simulink library "sm_wheel_loader_lib"  (R2025a)
settings: Solver=VariableStepAuto  StartTime=0.0  StopTime=10.0  RelTol=1e-3
undefined symbols (not defined in the file): AToTOrificeVector, BiPOrificeVector, boomHEArea, boomREArea, BToTOrificeVector, fluids, GRake, GToothL, GToothR, HMPST, HydFcnParams, logLoad, Position, PToAOrificeVector, PToBOrificeVector, RakeL, RakeR, testInput, Wheel_Loader, X, Y, Z
libraries: sm_lib x694, fl_lib x183, nesl_utility x74, SimscapeFluids_lib x62, sdl_lib x25, cvt_components_lib x25, simulink_extras x5, $bdroot x4, wheel_loader_contact_lib x4, ee_lib x2, SignalEditorBlockLib x1, batteryecm_lib x1
(part 14 of 26)

== system sm_wheel_loader_lib/Wheel Loader Vehicle/Load/Log/Bin ==
  Brick A : sm_lib/Body Elements/Brick Solid  BrickDimensions="[0.1 5.5  1]"  BrickDimensionsUnits=m  ExportEntireGeometry=on  InertiaType=CalculateFromGeometry  BasedOnType=Density  Density=1000  DensityUnits=kg/m^3  Mass=1  MassUnits=kg  CenterOfMass=[0 0 0]  CenterOfMassUnits=m  MomentsOfInertia=[1 1 1]  MomentsOfInertiaUnits=kg*m^2  ProductsOfInertia=[0 0 0]  ProductsOfInertiaUnits=kg*m^2  GraphicType=FromGeometry  MarkerShape=Sphere  MarkerSize=10  GraphicVisPropType=SimpleVisualProperties  GraphicDiffuseColor=[0.5 0.5 0.5]  GraphicOpacity=1.0  GraphicSpecularColor=[0.5 0.5 0.5 1.0]  GraphicAmbientColor=[0.15 0.15 0.15 1.0]  GraphicEmissiveColor=[0.0 0.0 0.0 1.0]  GraphicShininess=75  DoExposeReferenceFrame=on  SerializedFrames=<Frames/>
  Brick B : sm_lib/Body Elements/Brick Solid  BrickDimensions=[0.1 5.5 1]  BrickDimensionsUnits=m  ExportEntireGeometry=on  InertiaType=CalculateFromGeometry  BasedOnType=Density  Density=1000  DensityUnits=kg/m^3  Mass=1  MassUnits=kg  CenterOfMass=[0 0 0]  CenterOfMassUnits=m  MomentsOfInertia=[1 1 1]  MomentsOfInertiaUnits=kg*m^2  ProductsOfInertia=[0 0 0]  ProductsOfInertiaUnits=kg*m^2  GraphicType=FromGeometry  MarkerShape=Sphere  MarkerSize=10  GraphicVisPropType=SimpleVisualProperties  GraphicDiffuseColor=[0.5 0.5 0.5]  GraphicOpacity=1.0  GraphicSpecularColor=[0.5 0.5 0.5 1.0]  GraphicAmbientColor=[0.15 0.15 0.15 1.0]  GraphicEmissiveColor=[0.0 0.0 0.0 1.0]  GraphicShininess=75  DoExposeReferenceFrame=on  SerializedFrames=<Frames/>
  Transform Location Base : sm_lib/Frames and Transforms/Rigid Transform  RotationMethod=None  FollAlignAxisA=+X  BaseAlignAxisA=+Y  FollAlignAxisB=+Y  BaseAlignAxisB=+Z  RotationStandardAxis=+Z  RotationAngle=0.0  RotationAngleUnits=deg  RotationArbitraryAxis=[0 0 1]  RotationSequenceAxes=FollowerAxes  RotationSequence=XYX  RotationSequenceAngles=[0 0 0]  RotationSequenceAnglesUnits=deg  RotationMatrix=[1 0 0; 0 1 0; 0 0 1]  Quaternion=[1 0 0 0]  TranslationMethod=Cartesian  TranslationCartesianOffset=TranslationCartesianOffset  TranslationCartesianOffsetUnits=m  TranslationStandardAxis=+Z  TranslationStandardOffset=0  TranslationStandardOffsetUnits=m  TranslationROffset=0  TranslationROffsetUnits=m  TranslationThetaOffset=0  TranslationThetaOffsetUnits=deg  TranslationZOffset=0  TranslationZOffsetUnits=m
  Transform Orient Base : sm_lib/Frames and Transforms/Rigid Transform  RotationMethod=StandardAxis  FollAlignAxisA=+X  BaseAlignAxisA=+Y  FollAlignAxisB=+Y  BaseAlignAxisB=+Z  RotationStandardAxis=+Z  RotationAngle=RotationAngle  RotationAngleUnits=deg  RotationArbitraryAxis=[0 0 1]  RotationSequenceAxes=FollowerAxes  RotationSequence=XYX  RotationSequenceAngles=[0 0 0]  RotationSequenceAnglesUnits=deg  RotationMatrix=[1 0 0; 0 1 0; 0 0 1]  Quaternion=[1 0 0 0]  TranslationMethod=None  TranslationCartesianOffset=[0 0 0]  TranslationCartesianOffsetUnits=m  TranslationStandardAxis=+Z  TranslationStandardOffset=0  TranslationStandardOffsetUnits=m  TranslationROffset=0  TranslationROffsetUnits=m  TranslationThetaOffset=0  TranslationThetaOffsetUnits=deg  TranslationZOffset=0  TranslationZOffsetUnits=m
  Transform Plate A : sm_lib/Frames and Transforms/Rigid Transform  RotationMethod=StandardAxis  FollAlignAxisA=+X  BaseAlignAxisA=+Y  FollAlignAxisB=+Y  BaseAlignAxisB=+Z  RotationStandardAxis=+Y  RotationAngle=60  RotationAngleUnits=deg  RotationArbitraryAxis=[0 0 1]  RotationSequenceAxes=FollowerAxes  RotationSequence=XYX  RotationSequenceAngles=[0 0 0]  RotationSequenceAnglesUnits=deg  RotationMatrix=[1 0 0; 0 1 0; 0 0 1]  Quaternion=[1 0 0 0]  TranslationMethod=Cartesian  TranslationCartesianOffset="[0.45  0  0.5]"  TranslationCartesianOffsetUnits=m  TranslationStandardAxis=+Z  TranslationStandardOffset=0  TranslationStandardOffsetUnits=m  TranslationROffset=0  TranslationROffsetUnits=m  TranslationThetaOffset=0  TranslationThetaOffsetUnits=deg  TranslationZOffset=0  TranslationZOffsetUnits=m
  Transform Plate B : sm_lib/Frames and Transforms/Rigid Transform  RotationMethod=StandardAxis  FollAlignAxisA=+X  BaseAlignAxisA=+Y  FollAlignAxisB=+Y  BaseAlignAxisB=+Z  RotationStandardAxis=+Y  RotationAngle=-60  RotationAngleUnits=deg  RotationArbitraryAxis=[0 0 1]  RotationSequenceAxes=FollowerAxes  RotationSequence=XYX  RotationSequenceAngles=[0 0 0]  RotationSequenceAnglesUnits=deg  RotationMatrix=[1 0 0; 0 1 0; 0 0 1]  Quaternion=[1 0 0 0]  TranslationMethod=Cartesian  TranslationCartesianOffset="[-0.45  0  0.5]"  TranslationCartesianOffsetUnits=m  TranslationStandardAxis=+Z  TranslationStandardOffset=0  TranslationStandardOffsetUnits=m  TranslationROffset=0  TranslationROffsetUnits=m  TranslationThetaOffset=0  TranslationThetaOffsetUnits=deg  TranslationZOffset=0  TranslationZOffsetUnits=m
  A : PMIOPort  Side=Right
  W : PMIOPort  Port=2  Side=Left
  B : PMIOPort  Port=3  Side=Right
  connections:
  W/RConn1 -- Transform Location Base/LConn1
  Transform Orient Base/LConn1 -- Transform Location Base/RConn1
  A/RConn1 -- Brick A/LConn1
  Brick B/RConn1 -- Transform Plate B/RConn1
  Transform Plate A/RConn1 -- Brick A/RConn1
  Transform Plate A/LConn1 -- Transform Orient Base/RConn1 -- Transform Plate B/LConn1
  Brick B/LConn1 -- B/RConn1

== system sm_wheel_loader_lib/Wheel Loader Vehicle/Load/Log/Log ==
  Point Cloud Log L : sm_lib/Curves and Surfaces/Point Cloud  CoordinatesMatrix=[sin(linspace(0,24/25*2*pi,25))' cos(linspace(0,24/25*2*pi,25))' zeros(25,1)]*logLoad.rad  CoordinatesMatrixUnits=m  GraphicType=MarkerCloud  GraphicSphereRadius=1e-3  GraphicSphereRadiusUnits=m  GraphicVisPropType=SimpleVisualProperties  GraphicDiffuseColor=[0.5 0.5 0.5]  GraphicOpacity=1.0  GraphicSpecularColor=[0.5 0.5 0.5 1.0]  GraphicAmbientColor=[0.15 0.15 0.15 1.0]  GraphicEmissiveColor=[0.0 0.0 0.0 1.0]  GraphicShininess=75
  Point Cloud Log R : sm_lib/Curves and Surfaces/Point Cloud  CoordinatesMatrix=[sin(linspace(0,24/25*2*pi,25))' cos(linspace(0,24/25*2*pi,25))' zeros(25,1)]*logLoad.rad  CoordinatesMatrixUnits=m  GraphicType=MarkerCloud  GraphicSphereRadius=1e-3  GraphicSphereRadiusUnits=m  GraphicVisPropType=SimpleVisualProperties  GraphicDiffuseColor=[0.5 0.5 0.5]  GraphicOpacity=1.0  GraphicSpecularColor=[0.5 0.5 0.5 1.0]  GraphicAmbientColor=[0.15 0.15 0.15 1.0]  GraphicEmissiveColor=[0.0 0.0 0.0 1.0]  GraphicShininess=75
  Wooden Log : sm_lib/Body Elements/Cylindrical Solid  CylinderRadius=logLoad.rad  CylinderRadiusUnits=m  CylinderLength=logLoad.len  CylinderLengthUnits=m  ExportEntireGeometry=on  InertiaType=CalculateFromGeometry  BasedOnType=Density  Density=1000  DensityUnits=kg/m^3  Mass=50  MassUnits=kg  CenterOfMass=[0 0 0]  CenterOfMassUnits=m  MomentsOfInertia=[1 1 1]  MomentsOfInertiaUnits=kg*m^2  ProductsOfInertia=[0 0 0]  ProductsOfInertiaUnits=kg*m^2  GraphicType=FromGeometry  MarkerShape=Sphere  MarkerSize=10  GraphicVisPropType=SimpleVisualProperties  GraphicDiffuseColor=[0.9411765 0.73333335 0.5529412]  GraphicOpacity=1.0  GraphicSpecularColor=[0.5 0.5 0.5 1.0]  GraphicAmbientColor=[0.15 0.15 0.15 1.0]  GraphicEmissiveColor=[0.0 0.0 0.0 1.0]  GraphicShininess=75  DoExposeReferenceFrame=on  SerializedFrames=<Frames><Frame><Id>Frame1</Id><Value><Name>F</Name><Origin><Source>GeometricFeature</Source><FeatureName>top surface</FeatureName></Origin><PrimaryAxis><DefinedDirection>+Z</DefinedDirection><Source>ReferenceFrame</Source><SourceDirection>+Z</SourceDirection><FeatureName></FeatureName></PrimaryAxis><SecondaryAxis><DefinedDirection>+X</DefinedDirection><Source>ReferenceFrame</Source><SourceDirection>+X</SourceDirection><FeatureName></FeatureName></SecondaryAxis></Value></Frame><Frame><Id>Frame2</Id><Value><Name>B</Name><Origin><Source>GeometricFeature</Source><FeatureName>bottom surface</FeatureName></Origin><PrimaryAxis><DefinedDirection>+Z</DefinedDirection><Source>ReferenceFrame</Source><SourceDirection>+Z</SourceDirection><FeatureName></FeatureName></PrimaryAxis><SecondaryAxis><DefinedDirection>+X</DefinedDirection><Source>ReferenceFrame</Source><SourceDirection>+X</SourceDirection><FeatureName></FeatureName></SecondaryAxis></Value></Frame></Frames>
  Gdl : PMIOPort  Side=Left
  Gdr : PMIOPort  Port=2  Side=Left
  Gc : PMIOPort  Port=3  Side=Left
  R : PMIOPort  Port=4  Side=Right
  connections:
  Point Cloud Log R/LConn1 -- Wooden Log/LConn2
  Gc/RConn1 -- Wooden Log/RConn2
  Gdr/RConn1 -- Point Cloud Log R/RConn1
  Point Cloud Log L/RConn1 -- Gdl/RConn1
  Wooden Log/LConn1 -- Point Cloud Log L/LConn1
  R/RConn1 -- Wooden Log/RConn1

== system sm_wheel_loader_lib/Wheel Loader Vehicle/Steering Actuator/Actuator/Position ==
  p : Inport
  Abs : Abs  ZeroCross=off  SaturateOnIntegerOverflow=off
  Bus Selector : BusSelector  OutputSignals=Actuator.steeringAct.pos
  Cylindrical Steering Actuator : sm_lib/Joints/Cylindrical Joint  JointMode=Normal  CompositeWrenchDir=FollowerOnBase  CompositeWrenchFrame=BaseFrame  SenseConstraintForce=off  SenseConstraintTorque=off  SenseTotalForce=off  SenseTotalTorque=off  RzPositionTargetSpecify=off  RzPositionTargetPriority=High  RzPositionTargetValue=0  RzPositionTargetValueUnits=deg  RzVelocityTargetSpecify=off  RzVelocityTargetPriority=High  RzVelocityTargetValue=0  RzVelocityTargetValueUnits=deg/s  RzEquilibriumPosition=0  RzEquilibriumPositionUnits=deg  RzSpringStiffness=0  RzSpringStiffnessUnits=N*m/deg  RzDampingCoefficient=0  RzDampingCoefficientUnits=N*m/(deg/s)  RzLowerLimitSpecify=off  RzLowerLimitBound=-90  RzLowerLimitBoundUnits=deg  RzLowerLimitStiffness=1e4  RzLowerLimitStiffnessUnits=N*m/deg  RzLowerLimitDamping=10  RzLowerLimitDampingUnits=N*m/(deg/s)  RzLowerLimitTransitionRegionWidth=0.1  RzLowerLimitTransitionRegionWidthUnits=deg  RzUpperLimitSpecify=off  RzUpperLimitBound=90  RzUpperLimitBoundUnits=deg  RzUpperLimitStiffness=1e4  RzUpperLimitStiffnessUnits=N*m/deg  RzUpperLimitDamping=10  RzUpperLimitDampingUnits=N*m/(deg/s)  RzUpperLimitTransitionRegionWidth=0.1  RzUpperLimitTransitionRegionWidthUnits=deg  RzTorqueActuationMode=NoTorque  RzMotionActuationMode=ComputedMotion  RzSensePosition=off  RzSenseVelocity=off  RzSenseAcceleration=off  RzSenseTorqueForce=off  RzSenseLowerLimitTorqueForce=off  RzSenseUpperLimitTorqueForce=off  PzPositionTargetSpecify=on  PzPositionTargetPriority=High  PzPositionTargetValue=testInput.Active.Steer.p(1)*1000  PzPositionTargetValueUnits=mm  PzVelocityTargetSpecify=off  PzVelocityTargetPriority=High  PzVelocityTargetValue=0  PzVelocityTargetValueUnits=m/s  PzEquilibriumPosition=0  PzEquilibriumPositionUnits=m  PzSpringStiffness=0  PzSpringStiffnessUnits=N/m  PzDampingCoefficient=HMPST.Linkage.Actuator.damping  PzDampingCoefficientUnits=N/(m/s)  PzLowerLimitSpecify=off  PzLowerLimitBound=-1  PzLowerLimitBoundUnits=m  PzLowerLimitStiffness=1e6  PzLowerLimitStiffnessUnits=N/m  PzLowerLimitDamping=1e3  PzLowerLimitDampingUnits=N/(m/s)  PzLowerLimitTransitionRegionWidth=1e-4  PzLowerLimitTransitionRegionWidthUnits=m  PzUpperLimitSpecify=off  PzUpperLimitBound=1  PzUpperLimitBoundUnits=m  PzUpperLimitStiffness=1e6  PzUpperLimitStiffnessUnits=N/m  PzUpperLimitDamping=1e3  PzUpperLimitDampingUnits=N/(m/s)  PzUpperLimitTransitionRegionWidth=1e-4  PzUpperLimitTransitionRegionWidthUnits=m  PzTorqueActuationMode=ComputedTorque  PzMotionActuationMode=InputMotion  PzSensePosition=on  PzSenseVelocity=on  PzSenseAcceleration=off  PzSenseTorqueForce=on  PzSenseLowerLimitTorqueForce=off  PzSenseUpperLimitTorqueForce=off
  Gain : Gain
  PS-Simulink Converter : nesl_utility/PS-Simulink Converter  PhysicalDomain=network_engine_domain  SubClassName=ps_output  LeftPortType=input  RightPortType=output  PseudoPeriodic=off  Frequencies=[]  VectorFormat=inherit  Unit=inherit  AffineConversion=off
  PS-Simulink Converter1 : nesl_utility/PS-Simulink Converter  PhysicalDomain=network_engine_domain  SubClassName=ps_output  LeftPortType=input  RightPortType=output  PseudoPeriodic=off  Frequencies=[]  VectorFormat=inherit  Unit=inherit  AffineConversion=off
  PS-Simulink Converter2 : nesl_utility/PS-Simulink Converter  PhysicalDomain=network_engine_domain  SubClassName=ps_output  LeftPortType=input  RightPortType=output  PseudoPeriodic=off  Frequencies=[]  VectorFormat=inherit  Unit=inherit  AffineConversion=off
  Product : Product
  Simulink-PS Converter : nesl_utility/Simulink-PS Converter  PhysicalDomain=network_engine_domain  SubClassName=ps_input  LeftPortType=input  RightPortType=output  PseudoPeriodic=off  Frequencies=[]  NoiseDistribution=none  NoiseParameters=[]  Unit=mm  AffineConversion=off  FilteringAndDerivatives=filter  SimscapeFilterOrder=2  InputFilterTimeConstant=0.01  UdotUserProvided=0
  Transfer Fcn : TransferFcn  Denominator=[0.01 1]
  R : PMIOPort  Side=Left
  B : PMIOPort  Port=2  Side=Left
  F : PMIOPort  Port=3  Side=Right
  Out Bus Element : Outport  PortName=m  Element=power
  Out Bus Element1 : Outport  PortName=m  Element=force
  Out Bus Element2 : Outport  PortName=m  Element=v
  Out Bus Element3 : Outport  PortName=m  Element=p
  wires:
  p/1 -> Bus Selector/1
  Gain/1 -> Simulink-PS Converter/1
  Bus Selector/1 -> Gain/1  "<pos>"
  PS-Simulink Converter1/1 -> Out Bus Element2/1, Product/1
  PS-Simulink Converter2/1 -> Out Bus Element3/1
  Product/1 -> Abs/1
  Abs/1 -> Out Bus Element/1
  PS-Simulink Converter/1 -> Transfer Fcn/1, Product/2
  Transfer Fcn/1 -> Out Bus Element1/1
  connections:
  Cylindrical Steering Actuator/RConn1 -- F/RConn1
  B/RConn1 -- Cylindrical Steering Actuator/LConn1
  Cylindrical Steering Actuator/RConn3 -- PS-Simulink Converter1/LConn1
  Cylindrical Steering Actuator/RConn2 -- PS-Simulink Converter2/LConn1
  Cylindrical Steering Actuator/RConn4 -- PS-Simulink Converter/LConn1
  Simulink-PS Converter/RConn1 -- Cylindrical Steering Actuator/LConn2

== system sm_wheel_loader_lib/Wheel Loader Vehicle/Steering Actuator/Actuator/Shaft ==
  p : Inport
  Abs : Abs  ZeroCross=off  SaturateOnIntegerOverflow=off
  Cylindrical Steering Actuator : sm_lib/Joints/Cylindrical Joint  JointMode=Normal  CompositeWrenchDir=FollowerOnBase  CompositeWrenchFrame=BaseFrame  SenseConstraintForce=off  SenseConstraintTorque=off  SenseTotalForce=off  SenseTotalTorque=off  RzPositionTargetSpecify=off  RzPositionTargetPriority=High  RzPositionTargetValue=0  RzPositionTargetValueUnits=deg  RzVelocityTargetSpecify=off  RzVelocityTargetPriority=High  RzVelocityTargetValue=0  RzVelocityTargetValueUnits=deg/s  RzEquilibriumPosition=0  RzEquilibriumPositionUnits=deg  RzSpringStiffness=0  RzSpringStiffnessUnits=N*m/deg  RzDampingCoefficient=0  RzDampingCoefficientUnits=N*m/(deg/s)  RzLowerLimitSpecify=off  RzLowerLimitBound=-90  RzLowerLimitBoundUnits=deg  RzLowerLimitStiffness=1e4  RzLowerLimitStiffnessUnits=N*m/deg  RzLowerLimitDamping=10  RzLowerLimitDampingUnits=N*m/(deg/s)  RzLowerLimitTransitionRegionWidth=0.1  RzLowerLimitTransitionRegionWidthUnits=deg  RzUpperLimitSpecify=off  RzUpperLimitBound=90  RzUpperLimitBoundUnits=deg  RzUpperLimitStiffness=1e4  RzUpperLimitStiffnessUnits=N*m/deg  RzUpperLimitDamping=10  RzUpperLimitDampingUnits=N*m/(deg/s)  RzUpperLimitTransitionRegionWidth=0.1  RzUpperLimitTransitionRegionWidthUnits=deg  RzTorqueActuationMode=NoTorque  RzMotionActuationMode=ComputedMotion  RzSensePosition=off  RzSenseVelocity=off  RzSenseAcceleration=off  RzSenseTorqueForce=off  RzSenseLowerLimitTorqueForce=off  RzSenseUpperLimitTorqueForce=off  PzPositionTargetSpecify=on  PzPositionTargetPriority=High  PzPositionTargetValue=testInput.Active.Steer.p(1)*1000  PzPositionTargetValueUnits=mm  PzVelocityTargetSpecify=off  PzVelocityTargetPriority=High  PzVelocityTargetValue=0  PzVelocityTargetValueUnits=m/s  PzEquilibriumPosition=0  PzEquilibriumPositionUnits=m  PzSpringStiffness=0  PzSpringStiffnessUnits=N/m  PzDampingCoefficient=HMPST.Linkage.Actuator.damping  PzDampingCoefficientUnits=N/(m/s)  PzLowerLimitSpecify=off  PzLowerLimitBound=-1  PzLowerLimitBoundUnits=m  PzLowerLimitStiffness=1e6  PzLowerLimitStiffnessUnits=N/m  PzLowerLimitDamping=1e3  PzLowerLimitDampingUnits=N/(m/s)  PzLowerLimitTransitionRegionWidth=1e-4  PzLowerLimitTransitionRegionWidthUnits=m  PzUpperLimitSpecify=off  PzUpperLimitBound=1  PzUpperLimitBoundUnits=m  PzUpperLimitStiffness=1e6  PzUpperLimitStiffnessUnits=N/m  PzUpperLimitDamping=1e3  PzUpperLimitDampingUnits=N/(m/s)  PzUpperLimitTransitionRegionWidth=1e-4  PzUpperLimitTransitionRegionWidthUnits=m  PzTorqueActuationMode=InputTorque  PzMotionActuationMode=ComputedMotion  PzSensePosition=on  PzSenseVelocity=on  PzSenseAcceleration=off  PzSenseTorqueForce=on  PzSenseLowerLimitTorqueForce=off  PzSenseUpperLimitTorqueForce=off
  MTRef : fl_lib/Mechanical/Translational Elements/Mechanical Translational Reference
  PS-Simulink Converter : nesl_utility/PS-Simulink Converter  PhysicalDomain=network_engine_domain  SubClassName=ps_output  LeftPortType=input  RightPortType=output  PseudoPeriodic=off  Frequencies=[]  VectorFormat=inherit  Unit=inherit  AffineConversion=off
  PS-Simulink Converter1 : nesl_utility/PS-Simulink Converter  PhysicalDomain=network_engine_domain  SubClassName=ps_output  LeftPortType=input  RightPortType=output  PseudoPeriodic=off  Frequencies=[]  VectorFormat=inherit  Unit=inherit  AffineConversion=off
  PS-Simulink Converter2 : nesl_utility/PS-Simulink Converter  PhysicalDomain=network_engine_domain  SubClassName=ps_output  LeftPortType=input  RightPortType=output  PseudoPeriodic=off  Frequencies=[]  VectorFormat=inherit  Unit=inherit  AffineConversion=off
  Product : Product
  Terminator : Terminator
  Transfer Fcn : TransferFcn  Denominator=[0.01 1]
  Translational Multibody Interface : fl_lib/Mechanical/Multibody Interfaces/Translational Multibody Interface
  R : PMIOPort  Side=Left
  B : PMIOPort  Port=2  Side=Left
  F : PMIOPort  Port=3  Side=Right
  Out Bus Element : Outport  PortName=m  Element=power
  Out Bus Element1 : Outport  PortName=m  Element=force
  Out Bus Element2 : Outport  PortName=m  Element=v
  Out Bus Element3 : Outport  PortName=m  Element=p
  wires:
  Transfer Fcn/1 -> Out Bus Element1/1
  PS-Simulink Converter/1 -> Product/2, Transfer Fcn/1
  Abs/1 -> Out Bus Element/1
  Product/1 -> Abs/1
  PS-Simulink Converter2/1 -> Out Bus Element3/1
  PS-Simulink Converter1/1 -> Product/1, Out Bus Element2/1
  p/1 -> Terminator/1
  connections:
  Cylindrical Steering Actuator/RConn4 -- PS-Simulink Converter/LConn1
  Cylindrical Steering Actuator/RConn2 -- PS-Simulink Converter2/LConn1
  Cylindrical Steering Actuator/RConn3 -- Translational Multibody Interface/RConn1 -- PS-Simulink Converter1/LConn1
  Translational Multibody Interface/LConn1 -- Cylindrical Steering Actuator/LConn2
  B/RConn1 -- Cylindrical Steering Actuator/LConn1
  Cylindrical Steering Actuator/RConn1 -- F/RConn1
  Translational Multibody Interface/LConn2 -- MTRef/LConn1
  R/RConn1 -- Translational Multibody Interface/RConn2

== system sm_wheel_loader_lib/Wheel Loader Vehicle/Actuators/Hydraulic/Implement/Bucket ==
  note: There are no actuators within the bucket implement.
  A : Inport
  Terminator : Terminator
  Impl : PMIOPort  Side=Right
  wires:
  A/1 -> Terminator/1

== system sm_wheel_loader_lib/Wheel Loader Vehicle/Actuators/Hydraulic/Implement/Grapple ==
  note: This is an abstract model of the toothbar cylinders that has a 1D mechnanical shaft as its interface.
  A : Inport
  Bus Selector4 : BusSelector  OutputSignals=leftToothbarAct.pos,rightToothbarAct.pos
  Damper ToothbarL : sdl_lib/Couplings & Drives/Springs & Dampers/Translational Damper  D=1e6 N*s/m  thermal_port=simscape.enum.thermaleffects.omit  thermal_mass=50 kJ/K  temperature_specify=off  temperature_priority=High  temperature=300 K  temperature_nominal_specify=off  temperature_nominal_value=1  temperature_nominal_unit=K
  Damper ToothbarR : sdl_lib/Couplings & Drives/Springs & Dampers/Translational Damper  D=1e6 N*s/m  thermal_port=simscape.enum.thermaleffects.omit  thermal_mass=50 kJ/K  temperature_specify=off  temperature_priority=High  temperature=300 K  temperature_nominal_specify=off  temperature_nominal_value=1  temperature_nominal_unit=K
  MTRef ToothbarL : fl_lib/Mechanical/Translational Elements/Mechanical Translational Reference
  MTRef ToothbarR : fl_lib/Mechanical/Translational Elements/Mechanical Translational Reference
  Simscape Bus : SimscapeBus  HierarchyStrings=RakeL;RakeR
  Simulink-PS Converter4 : nesl_utility/Simulink-PS Converter  PhysicalDomain=network_engine_domain  SubClassName=ps_input  LeftPortType=input  RightPortType=output  PseudoPeriodic=off  Frequencies=[]  NoiseDistribution=none  NoiseParameters=[]  Unit=mm/s  AffineConversion=off  FilteringAndDerivatives=filter  SimscapeFilterOrder=1  InputFilterTimeConstant=0.01  UdotUserProvided=0
  Simulink-PS Converter5 : nesl_utility/Simulink-PS Converter  PhysicalDomain=network_engine_domain  SubClassName=ps_input  LeftPortType=input  RightPortType=output  PseudoPeriodic=off  Frequencies=[]  NoiseDistribution=none  NoiseParameters=[]  Unit=mm/s  AffineConversion=off  FilteringAndDerivatives=filter  SimscapeFilterOrder=1  InputFilterTimeConstant=0.01  UdotUserProvided=0
  Spring ToothbarL : fl_lib/Mechanical/Translational Elements/Translational Spring  spr_rate=1e7 N/m  v_specify=off  v_priority=None  v=0 m/s  v_nominal_specify=off  v_nominal_value=1  v_nominal_unit=m/s  f_specify=off  f_priority=None  f=0 N  f_nominal_specify=off  f_nominal_value=1  f_nominal_unit=N  x_specify=off  x_priority=High  x=0 m  x_nominal_specify=off  x_nominal_value=1  x_nominal_unit=m
  Spring ToothbarR : fl_lib/Mechanical/Translational Elements/Translational Spring  spr_rate=1e7 N/m  v_specify=off  v_priority=None  v=0 m/s  v_nominal_specify=off  v_nominal_value=1  v_nominal_unit=m/s  f_specify=off  f_priority=None  f=0 N  f_nominal_specify=off  f_nominal_value=1  f_nominal_unit=N  x_specify=off  x_priority=High  x=0 m  x_nominal_specify=off  x_nominal_value=1  x_nominal_unit=m
  Transfer Fcn4 : TransferFcn  Numerator=[1 0]  Denominator=[0.1 1]
  Transfer Fcn5 : TransferFcn  Numerator=[1 0]  Denominator=[0.1 1]
  Velocity Source ToothbarL : fl_lib/Mechanical/Mechanical Sources/Ideal Translational Velocity Source
  Velocity Source ToothbarR : fl_lib/Mechanical/Mechanical Sources/Ideal Translational Velocity Source
  Impl : PMIOPort  Side=Right
  wires:
  Bus Selector4/1 -> Transfer Fcn4/1  "<pos>"
  Transfer Fcn5/1 -> Simulink-PS Converter5/1
  Transfer Fcn4/1 -> Simulink-PS Converter4/1
  Bus Selector4/2 -> Transfer Fcn5/1  "<pos>"
  A/1 -> Bus Selector4/1
  connections:
  Velocity Source ToothbarL/RConn1 -- Simulink-PS Converter4/RConn1
  Velocity Source ToothbarR/RConn1 -- Simulink-PS Converter5/RConn1
  Velocity Source ToothbarR/LConn1 -- Damper ToothbarR/RConn1 -- Spring ToothbarR/RConn1
  MTRef ToothbarR/LConn1 -- Velocity Source ToothbarR/RConn2
  Spring ToothbarR/LConn1 -- Damper ToothbarR/LConn1 -- Simscape Bus/LConn2
  Spring ToothbarL/LConn1 -- Damper ToothbarL/LConn1 -- Simscape Bus/LConn1
  Velocity Source ToothbarL/LConn1 -- Spring ToothbarL/RConn1 -- Damper ToothbarL/RConn1
  MTRef ToothbarL/LConn1 -- Velocity Source ToothbarL/RConn2
  Impl/RConn1 -- Simscape Bus/RConn1

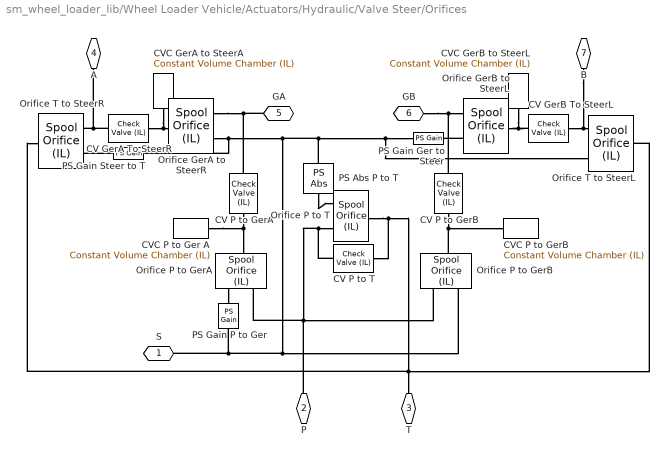
== system sm_wheel_loader_lib/Wheel Loader Vehicle/Actuators/Hydraulic/Valve Steer/Orifices ==
  CV GerA To SteerR : SimscapeFluids_lib/Isothermal Liquid/Valves & Orifices/Directional Control Valves/Check Valve (IL)  opening_spec=2*(fluids.isothermal_liquid.valves_orifices.enum.opening_spec.linear)-1  pressure_control_spec=fluids.isothermal_liquid.valves_orifices.enum.pressure_control_spec.dp  p_crack_differential=HydFcnParams.checkValves.crackingPrDiff bar  p_crack_gauge=0.1 MPa  press_max_differential=HydFcnParams.checkValves.maxOpeningPrDiff bar  press_max_gauge=0.2 MPa  area_max=HydFcnParams.checkValves.maxOpeningArea mm^2  area_leak="HydFcnParams.checkValves.leakageArea  mm^2"  p_diff_TLU=[0.01 : 0.01 : 0.1] MPa  valve_area_TLU=[1e-10, 1e-05, 2e-05, 3e-05, 4e-05, 5e-05, 6e-05, 7.5e-05, 8.5e-05, .0001] m^2  vol_flow_TLU=[.000358, .045, .11, .191, .284, .39, .505, .63, .764, .905] .* 1e-3 m^3/s  area=inf m^2  Cd=HydFcnParams.checkValves.dischargeCoef  Re_c=HydFcnParams.checkValves.critReynoldsNmbr  smoothing_factor=HydFcnParams.checkValves.smoothingFactor  pressure_recovery=simscape.enum.onoff.off  opening_dynamics=simscape.enum.onoff.off  tau=0.1 s
      settings: InternalSimscapePortConfiguration="{\"Bottom\":[],\"Left\":[{\"id\":\"A\",\"label\":\"A\",\"type\":\"foundation.isothermal_liquid.isothermal_liquid\"}],\"Right\":[{\"id\":\"B\",\"label\":\"B\",\"type\":\"foundation.isothermal_liquid.isothermal_liquid\"}],\"Top\":[]}"
  CV GerB To SteerL : SimscapeFluids_lib/Isothermal Liquid/Valves & Orifices/Directional Control Valves/Check Valve (IL)  opening_spec=2*(fluids.isothermal_liquid.valves_orifices.enum.opening_spec.linear)-1  pressure_control_spec=fluids.isothermal_liquid.valves_orifices.enum.pressure_control_spec.dp  p_crack_differential=HydFcnParams.checkValves.crackingPrDiff bar  p_crack_gauge=0.1 MPa  press_max_differential=HydFcnParams.checkValves.maxOpeningPrDiff bar  press_max_gauge=0.2 MPa  area_max=HydFcnParams.checkValves.maxOpeningArea mm^2  area_leak="HydFcnParams.checkValves.leakageArea  mm^2"  p_diff_TLU=[0.01 : 0.01 : 0.1] MPa  valve_area_TLU=[1e-10, 1e-05, 2e-05, 3e-05, 4e-05, 5e-05, 6e-05, 7.5e-05, 8.5e-05, .0001] m^2  vol_flow_TLU=[.000358, .045, .11, .191, .284, .39, .505, .63, .764, .905] .* 1e-3 m^3/s  area=inf m^2  Cd=HydFcnParams.checkValves.dischargeCoef  Re_c=HydFcnParams.checkValves.critReynoldsNmbr  smoothing_factor=HydFcnParams.checkValves.smoothingFactor  pressure_recovery=simscape.enum.onoff.off  opening_dynamics=simscape.enum.onoff.off  tau=0.1 s
      settings: InternalSimscapePortConfiguration="{\"Bottom\":[],\"Left\":[{\"id\":\"A\",\"label\":\"A\",\"type\":\"foundation.isothermal_liquid.isothermal_liquid\"}],\"Right\":[{\"id\":\"B\",\"label\":\"B\",\"type\":\"foundation.isothermal_liquid.isothermal_liquid\"}],\"Top\":[]}"
  CV P to GerA : SimscapeFluids_lib/Isothermal Liquid/Valves & Orifices/Directional Control Valves/Check Valve (IL)  opening_spec=2*(fluids.isothermal_liquid.valves_orifices.enum.opening_spec.linear)-1  pressure_control_spec=fluids.isothermal_liquid.valves_orifices.enum.pressure_control_spec.dp  p_crack_differential=HydFcnParams.checkValves.crackingPrDiff bar  p_crack_gauge=0.1 MPa  press_max_differential=HydFcnParams.checkValves.maxOpeningPrDiff bar  press_max_gauge=0.2 MPa  area_max=HydFcnParams.checkValves.maxOpeningArea mm^2  area_leak="HydFcnParams.checkValves.leakageArea  mm^2"  p_diff_TLU=[0.01 : 0.01 : 0.1] MPa  valve_area_TLU=[1e-10, 1e-05, 2e-05, 3e-05, 4e-05, 5e-05, 6e-05, 7.5e-05, 8.5e-05, .0001] m^2  vol_flow_TLU=[.000358, .045, .11, .191, .284, .39, .505, .63, .764, .905] .* 1e-3 m^3/s  area=inf m^2  Cd=HydFcnParams.checkValves.dischargeCoef  Re_c=HydFcnParams.checkValves.critReynoldsNmbr  smoothing_factor=HydFcnParams.checkValves.smoothingFactor  pressure_recovery=simscape.enum.onoff.off  opening_dynamics=simscape.enum.onoff.off  tau=0.1 s
      settings: InternalSimscapePortConfiguration="{\"Bottom\":[],\"Left\":[{\"id\":\"A\",\"label\":\"A\",\"type\":\"foundation.isothermal_liquid.isothermal_liquid\"}],\"Right\":[{\"id\":\"B\",\"label\":\"B\",\"type\":\"foundation.isothermal_liquid.isothermal_liquid\"}],\"Top\":[]}"
  CV P to GerB : SimscapeFluids_lib/Isothermal Liquid/Valves & Orifices/Directional Control Valves/Check Valve (IL)  opening_spec=2*(fluids.isothermal_liquid.valves_orifices.enum.opening_spec.linear)-1  pressure_control_spec=fluids.isothermal_liquid.valves_orifices.enum.pressure_control_spec.dp  p_crack_differential=HydFcnParams.checkValves.crackingPrDiff bar  p_crack_gauge=0.1 MPa  press_max_differential=HydFcnParams.checkValves.maxOpeningPrDiff bar  press_max_gauge=0.2 MPa  area_max=HydFcnParams.checkValves.maxOpeningArea mm^2  area_leak="HydFcnParams.checkValves.leakageArea  mm^2"  p_diff_TLU=[0.01 : 0.01 : 0.1] MPa  valve_area_TLU=[1e-10, 1e-05, 2e-05, 3e-05, 4e-05, 5e-05, 6e-05, 7.5e-05, 8.5e-05, .0001] m^2  vol_flow_TLU=[.000358, .045, .11, .191, .284, .39, .505, .63, .764, .905] .* 1e-3 m^3/s  area=inf m^2  Cd=HydFcnParams.checkValves.dischargeCoef  Re_c=HydFcnParams.checkValves.critReynoldsNmbr  smoothing_factor=HydFcnParams.checkValves.smoothingFactor  pressure_recovery=simscape.enum.onoff.off  opening_dynamics=simscape.enum.onoff.off  tau=0.1 s
      settings: InternalSimscapePortConfiguration="{\"Bottom\":[],\"Left\":[{\"id\":\"A\",\"label\":\"A\",\"type\":\"foundation.isothermal_liquid.isothermal_liquid\"}],\"Right\":[{\"id\":\"B\",\"label\":\"B\",\"type\":\"foundation.isothermal_liquid.isothermal_liquid\"}],\"Top\":[]}"
  CV P to T : SimscapeFluids_lib/Isothermal Liquid/Valves & Orifices/Directional Control Valves/Check Valve (IL)  opening_spec=2*(fluids.isothermal_liquid.valves_orifices.enum.opening_spec.linear)-1  pressure_control_spec=fluids.isothermal_liquid.valves_orifices.enum.pressure_control_spec.dp  p_crack_differential=HydFcnParams.checkValves.crackingPrDiff bar  p_crack_gauge=0.1 MPa  press_max_differential=HydFcnParams.checkValves.maxOpeningPrDiff bar  press_max_gauge=0.2 MPa  area_max=HydFcnParams.checkValves.maxOpeningArea mm^2  area_leak="HydFcnParams.checkValves.leakageArea  mm^2"  p_diff_TLU=[0.01 : 0.01 : 0.1] MPa  valve_area_TLU=[1e-10, 1e-05, 2e-05, 3e-05, 4e-05, 5e-05, 6e-05, 7.5e-05, 8.5e-05, .0001] m^2  vol_flow_TLU=[.000358, .045, .11, .191, .284, .39, .505, .63, .764, .905] .* 1e-3 m^3/s  area=inf m^2  Cd=HydFcnParams.checkValves.dischargeCoef  Re_c=HydFcnParams.checkValves.critReynoldsNmbr  smoothing_factor=HydFcnParams.checkValves.smoothingFactor  pressure_recovery=simscape.enum.onoff.off  opening_dynamics=simscape.enum.onoff.off  tau=0.1 s
      settings: InternalSimscapePortConfiguration="{\"Bottom\":[],\"Left\":[{\"id\":\"A\",\"label\":\"A\",\"type\":\"foundation.isothermal_liquid.isothermal_liquid\"}],\"Right\":[{\"id\":\"B\",\"label\":\"B\",\"type\":\"foundation.isothermal_liquid.isothermal_liquid\"}],\"Top\":[]}"
  CVC GerA to SteerA : fl_lib/Isothermal Liquid/Elements/Constant Volume Chamber (IL)  volume=HydFcnParams.steerValve.CVChamberVol mm^3  p_I_specify=off  p_I_priority=High  p_I=0.101325 MPa  p_I_nominal_specify=off  p_I_nominal_value=1  p_I_nominal_unit=MPa
      settings: InternalSimscapePortConfiguration="{\"Bottom\":[],\"Left\":[{\"id\":\"A\",\"label\":\"A\",\"type\":\"foundation.isothermal_liquid.isothermal_liquid\"}],\"Right\":[],\"Top\":[]}"
  CVC GerB to SteerL : fl_lib/Isothermal Liquid/Elements/Constant Volume Chamber (IL)  volume=HydFcnParams.steerValve.CVChamberVol mm^3  p_I_specify=off  p_I_priority=High  p_I=0.101325 MPa  p_I_nominal_specify=off  p_I_nominal_value=1  p_I_nominal_unit=MPa
      settings: InternalSimscapePortConfiguration="{\"Bottom\":[],\"Left\":[{\"id\":\"A\",\"label\":\"A\",\"type\":\"foundation.isothermal_liquid.isothermal_liquid\"}],\"Right\":[],\"Top\":[]}"
  CVC P to Ger A : fl_lib/Isothermal Liquid/Elements/Constant Volume Chamber (IL)  volume=HydFcnParams.steerValve.CVChamberVol mm^3  p_I_specify=off  p_I_priority=High  p_I=0.101325 MPa  p_I_nominal_specify=off  p_I_nominal_value=1  p_I_nominal_unit=MPa
      settings: InternalSimscapePortConfiguration="{\"Bottom\":[],\"Left\":[{\"id\":\"A\",\"label\":\"A\",\"type\":\"foundation.isothermal_liquid.isothermal_liquid\"}],\"Right\":[],\"Top\":[]}"
  CVC P to GerB : fl_lib/Isothermal Liquid/Elements/Constant Volume Chamber (IL)  volume=HydFcnParams.steerValve.CVChamberVol mm^3  p_I_specify=off  p_I_priority=High  p_I=0.101325 MPa  p_I_nominal_specify=off  p_I_nominal_value=1  p_I_nominal_unit=MPa
      settings: InternalSimscapePortConfiguration="{\"Bottom\":[],\"Left\":[{\"id\":\"A\",\"label\":\"A\",\"type\":\"foundation.isothermal_liquid.isothermal_liquid\"}],\"Right\":[],\"Top\":[]}"
  Orifice GerA to SteerR : SimscapeFluids_lib/Isothermal Liquid/Valves & Orifices/Orifices/Spool Orifice (IL)  orifice_spec=fluids.isothermal_liquid.valves_orifices.orifices.enum.spool_orifice.round_hole  diameter_hole=5 mm  num_hole=6  width=0.01 m  del_S_max=5e-3 m  S_min=0 m  open_orientation=fluids.isothermal_liquid.valves_orifices.enum.spool_orientation.positive  flow_force_spec=false  clearance=1e-5 m  area_leak=1e-10 m^2  area=inf m^2  Cd=0.64  Re_c=150  smoothing_factor=0.01  pressure_recovery=false
      settings: InternalSimscapePortConfiguration="{\"Bottom\":[],\"Left\":[{\"id\":\"S\",\"label\":\"S\",\"type\":\"input\"},{\"id\":\"A\",\"label\":\"A\",\"type\":\"foundation.isothermal_liquid.isothermal_liquid\"}],\"Right\":[{\"id\":\"B\",\"label\":\"B\",\"type\":\"foundation.isothermal_liquid.isothermal_liquid\"}],\"Top\":[]}"
  Orifice GerB to SteerL : SimscapeFluids_lib/Isothermal Liquid/Valves & Orifices/Orifices/Spool Orifice (IL)  orifice_spec=fluids.isothermal_liquid.valves_orifices.orifices.enum.spool_orifice.round_hole  diameter_hole=5 mm  num_hole=6  width=0.01 m  del_S_max=5e-3 m  S_min=0 m  open_orientation=fluids.isothermal_liquid.valves_orifices.enum.spool_orientation.positive  flow_force_spec=false  clearance=1e-5 m  area_leak=1e-10 m^2  area=inf m^2  Cd=0.64  Re_c=150  smoothing_factor=0.01  pressure_recovery=false
      settings: InternalSimscapePortConfiguration="{\"Bottom\":[],\"Left\":[{\"id\":\"S\",\"label\":\"S\",\"type\":\"input\"},{\"id\":\"A\",\"label\":\"A\",\"type\":\"foundation.isothermal_liquid.isothermal_liquid\"}],\"Right\":[{\"id\":\"B\",\"label\":\"B\",\"type\":\"foundation.isothermal_liquid.isothermal_liquid\"}],\"Top\":[]}"
  Orifice P to GerA : SimscapeFluids_lib/Isothermal Liquid/Valves & Orifices/Orifices/Spool Orifice (IL)  orifice_spec=fluids.isothermal_liquid.valves_orifices.orifices.enum.spool_orifice.round_hole  diameter_hole=5 mm  num_hole=6  width=0.01 m  del_S_max=5e-3 m  S_min=0 m  open_orientation=fluids.isothermal_liquid.valves_orifices.enum.spool_orientation.positive  flow_force_spec=false  clearance=1e-5 m  area_leak=1e-10 m^2  area=inf m^2  Cd=0.64  Re_c=150  smoothing_factor=0.01  pressure_recovery=false
      settings: InternalSimscapePortConfiguration="{\"Bottom\":[],\"Left\":[{\"id\":\"S\",\"label\":\"S\",\"type\":\"input\"},{\"id\":\"A\",\"label\":\"A\",\"type\":\"foundation.isothermal_liquid.isothermal_liquid\"}],\"Right\":[{\"id\":\"B\",\"label\":\"B\",\"type\":\"foundation.isothermal_liquid.isothermal_liquid\"}],\"Top\":[]}"
  Orifice P to GerB : SimscapeFluids_lib/Isothermal Liquid/Valves & Orifices/Orifices/Spool Orifice (IL)  orifice_spec=fluids.isothermal_liquid.valves_orifices.orifices.enum.spool_orifice.round_hole  diameter_hole=5 mm  num_hole=6  width=0.01 m  del_S_max=5e-3 m  S_min=0 m  open_orientation=fluids.isothermal_liquid.valves_orifices.enum.spool_orientation.positive  flow_force_spec=false  clearance=1e-5 m  area_leak=1e-10 m^2  area=inf m^2  Cd=0.64  Re_c=150  smoothing_factor=0.01  pressure_recovery=false
      settings: InternalSimscapePortConfiguration="{\"Bottom\":[],\"Left\":[{\"id\":\"S\",\"label\":\"S\",\"type\":\"input\"},{\"id\":\"A\",\"label\":\"A\",\"type\":\"foundation.isothermal_liquid.isothermal_liquid\"}],\"Right\":[{\"id\":\"B\",\"label\":\"B\",\"type\":\"foundation.isothermal_liquid.isothermal_liquid\"}],\"Top\":[]}"
  Orifice P to T : SimscapeFluids_lib/Isothermal Liquid/Valves & Orifices/Orifices/Spool Orifice (IL)  orifice_spec=fluids.isothermal_liquid.valves_orifices.orifices.enum.spool_orifice.round_hole  diameter_hole=5 mm  num_hole=6  width=0.01 m  del_S_max=5e-3 m  S_min=5 mm  open_orientation=fluids.isothermal_liquid.valves_orifices.enum.spool_orientation.negative  flow_force_spec=false  clearance=1e-5 m  area_leak=1e-8 m^2  area=inf m^2  Cd=0.64  Re_c=150  smoothing_factor=0.01  pressure_recovery=false
      settings: InternalSimscapePortConfiguration="{\"Bottom\":[],\"Left\":[{\"id\":\"S\",\"label\":\"S\",\"type\":\"input\"},{\"id\":\"A\",\"label\":\"A\",\"type\":\"foundation.isothermal_liquid.isothermal_liquid\"}],\"Right\":[{\"id\":\"B\",\"label\":\"B\",\"type\":\"foundation.isothermal_liquid.isothermal_liquid\"}],\"Top\":[]}"
  Orifice T to SteerL : SimscapeFluids_lib/Isothermal Liquid/Valves & Orifices/Orifices/Spool Orifice (IL)  orifice_spec=fluids.isothermal_liquid.valves_orifices.orifices.enum.spool_orifice.round_hole  diameter_hole=5 mm  num_hole=6  width=0.01 m  del_S_max=5e-3 m  S_min=0 m  open_orientation=fluids.isothermal_liquid.valves_orifices.enum.spool_orientation.positive  flow_force_spec=false  clearance=1e-5 m  area_leak=1e-10 m^2  area=inf m^2  Cd=0.64  Re_c=150  smoothing_factor=0.01  pressure_recovery=false
      settings: InternalSimscapePortConfiguration="{\"Bottom\":[],\"Left\":[{\"id\":\"S\",\"label\":\"S\",\"type\":\"input\"},{\"id\":\"A\",\"label\":\"A\",\"type\":\"foundation.isothermal_liquid.isothermal_liquid\"}],\"Right\":[{\"id\":\"B\",\"label\":\"B\",\"type\":\"foundation.isothermal_liquid.isothermal_liquid\"}],\"Top\":[]}"
  Orifice T to SteerR : SimscapeFluids_lib/Isothermal Liquid/Valves & Orifices/Orifices/Spool Orifice (IL)  orifice_spec=fluids.isothermal_liquid.valves_orifices.orifices.enum.spool_orifice.round_hole  diameter_hole=5 mm  num_hole=6  width=0.01 m  del_S_max=5e-3 m  S_min=0 m  open_orientation=fluids.isothermal_liquid.valves_orifices.enum.spool_orientation.positive  flow_force_spec=false  clearance=1e-5 m  area_leak=1e-10 m^2  area=inf m^2  Cd=0.64  Re_c=150  smoothing_factor=0.01  pressure_recovery=false
      settings: InternalSimscapePortConfiguration="{\"Bottom\":[],\"Left\":[{\"id\":\"S\",\"label\":\"S\",\"type\":\"input\"},{\"id\":\"A\",\"label\":\"A\",\"type\":\"foundation.isothermal_liquid.isothermal_liquid\"}],\"Right\":[{\"id\":\"B\",\"label\":\"B\",\"type\":\"foundation.isothermal_liquid.isothermal_liquid\"}],\"Top\":[]}"
  PS Abs P to T : fl_lib/Physical Signals/Nonlinear Operators/PS Abs  ZeroCross=true
      settings: InternalSimscapePortConfiguration="{\"Bottom\":[],\"Left\":[{\"id\":\"I\",\"label\":\"\",\"type\":\"input\"}],\"Right\":[{\"id\":\"O\",\"label\":\"\",\"type\":\"output\"}],\"Top\":[]}"
  PS Gain Ger to Steer : fl_lib/Physical Signals/Functions/PS Gain  gain=-1
  PS Gain P to Ger : fl_lib/Physical Signals/Functions/PS Gain  gain=-1
  PS Gain Steer to T : fl_lib/Physical Signals/Functions/PS Gain  gain=-1
  S : PMIOPort  Side=Left
  P : PMIOPort  Port=2  Side=Left
  T : PMIOPort  Port=3  Side=Left
  A : PMIOPort  Port=4  Side=Right
  GA : PMIOPort  Port=5  Side=Right
  GB : PMIOPort  Port=6  Side=Right
  B : PMIOPort  Port=7  Side=Right
  connections:
  CVC P to Ger A/LConn1 -- CV P to GerA/LConn1 -- Orifice P to GerA/RConn1
  B/RConn1 -- Orifice T to SteerL/LConn2 -- CV GerB To SteerL/RConn1
  CV GerA To SteerR/RConn1 -- A/RConn1 -- Orifice T to SteerR/LConn2
  CV P to T/LConn1 -- Orifice P to T/RConn1 -- T/RConn1 -- Orifice T to SteerR/RConn1 -- Orifice T to SteerL/RConn1
  PS Abs P to T/RConn1 -- Orifice P to T/LConn1
  Orifice GerA to SteerR/LConn1 -- PS Gain Steer to T/LConn1 -- PS Abs P to T/LConn1 -- Orifice T to SteerL/LConn1 -- PS Gain Ger to Steer/LConn1 -- S/RConn1 -- PS Gain P to Ger/LConn1 -- Orifice P to GerB/LConn1
  Orifice P to GerA/LConn1 -- PS Gain P to Ger/RConn1
  PS Gain Steer to T/RConn1 -- Orifice T to SteerR/LConn1
  Orifice GerB to SteerL/LConn1 -- PS Gain Ger to Steer/RConn1
  CVC GerA to SteerA/LConn1 -- CV GerA To SteerR/LConn1 -- Orifice GerA to SteerR/RConn1
  Orifice GerB to SteerL/RConn1 -- CV GerB To SteerL/LConn1 -- CVC GerB to SteerL/LConn1
  Orifice P to GerB/RConn1 -- CV P to GerB/LConn1 -- CVC P to GerB/LConn1
  P/RConn1 -- Orifice P to GerB/LConn2 -- CV P to T/RConn1 -- Orifice P to T/LConn2 -- Orifice P to GerA/LConn2
  GB/RConn1 -- CV P to GerB/RConn1 -- Orifice GerB to SteerL/LConn2
  Orifice GerA to SteerR/LConn2 -- CV P to GerA/RConn1 -- GA/RConn1

== system sm_wheel_loader_lib/Wheel Loader Vehicle/Actuators/Hydraulic/Valve Steer/qSleeve to xSpool ==
  PS Dead Zone : fl_lib/Physical Signals/Nonlinear Operators/PS Dead Zone  upper_limit=HydFcnParams.steerValve.deadZoneUpperLim rad  lower_limit=HydFcnParams.steerValve.deadZoneLowerLim rad  ZeroCross=true
      settings: InternalSimscapePortConfiguration="{\"Bottom\":[],\"Left\":[{\"id\":\"I\",\"label\":\"\",\"type\":\"input\"}],\"Right\":[{\"id\":\"O\",\"label\":\"\",\"type\":\"output\"}],\"Top\":[]}"
  PS Gain : fl_lib/Physical Signals/Functions/PS Gain  gain=HydFcnParams.steerValve.relAngleGain mm/rad
  PS Saturation : fl_lib/Physical Signals/Nonlinear Operators/PS Saturation  upper_limit=HydFcnParams.steerValve.spoolPosMax mm  lower_limit=HydFcnParams.steerValve.spoolPosMin mm  ZeroCross=true
  q : PMIOPort  Side=Left
  S : PMIOPort  Port=2  Side=Right
  connections:
  PS Saturation/LConn1 -- PS Gain/RConn1
  PS Saturation/RConn1 -- S/RConn1
  q/RConn1 -- PS Dead Zone/LConn1
  PS Dead Zone/RConn1 -- PS Gain/LConn1

== system sm_wheel_loader_lib/Wheel Loader Vehicle/Actuators/Hydraulic/Valves Linkage/Flow Divider ==
  note: Flow Divider
      | The flow divider splits the pump flow between the tilt and lift valves relative to the pressure differential between the two functions. This is used to maintain consistent actuator velocity when one or both functions are active as well as balance the velocities of the actuators - response of tilt to X joystick input should be similar to response of lift.
      |
      | The fixed orifices set the flow rate difference to achieve the balanced velocity. The variable orifices and actuator maintain consistent velocity.
      |
      | Monitor the flow rate from the pump against the flow through these orifices and the actuator speeds and pressures to check the impact of changes.
  Double-Acting Servo Valve Actuator (IL) : SimscapeFluids_lib/Isothermal Liquid/Valves & Orifices/Valve Actuators & Forces/Double-Acting Servo Valve Actuator (IL)  spool_area=1e-4 m^2  stroke=5e-3 m  stiff_coeff=HydFcnParams.flowDivider.actuatorStiffness N/m  damping_coeff=150 N*s/m  hardstop_model=simscape.enum.hardstop.smooth  stiff_coeff_hs=1e10 N/m  damping_coeff_hs=150 N*s/m  transition=0.1 mm  coeff_rest=0.7  v_tol=0.001 m/s  f_tol=0.001 N  x0=0 m  dynamic_compressibility=true  p0_A=10 bar  p0_B=10 bar  p_nominal_A=0.101325 MPa  p_nominal_B=0.101325 MPa
      settings: InternalSimscapePortConfiguration="{\"Bottom\":[],\"Left\":[{\"id\":\"A\",\"label\":\"A\",\"type\":\"foundation.isothermal_liquid.isothermal_liquid\"},{\"id\":\"B\",\"label\":\"B\",\"type\":\"foundation.isothermal_liquid.isothermal_liquid\"}],\"Right\":[{\"id\":\"S\",\"label\":\"S\",\"type\":\"output\"}],\"Top\":[]}"
  Fixed Orifice Lift : SimscapeFluids_lib/Isothermal Liquid/Valves & Orifices/Orifices/Orifice (IL)  orifice_type=foundation.enum.constant_variable.constant  constant_orifice_spec=fluids.isothermal_liquid.valves_orifices.orifices.enum.constant_orifice_spec.area  variable_orifice_spec=fluids.isothermal_liquid.valves_orifices.orifices.enum.orifice_spec.linear  orifice_area_constant=HydFcnParams.flowDivider.liftFixedOrificeArea mm^2  p_diff_TLU_constant=[-4, -3, -2, -1, -.5, 0, .5, 1, 2, 3, 4] MPa  vol_flow_TLU_constant=[-2.44, -2.12, -1.68, -1.22, -.84, 0, .85, 1.21, 1.7, 2.09, 2.41] .* 1e-3 m^3/s  S_min=0 m  del_S=5e-3 m  open_orientation=fluids.isothermal_liquid.valves_orifices.orifices.enum.orifice_orientation.positive  area_max=HydFcnParams.flowDivider.tiltMaxOrificeArea mm^2  area_leak=1e-10 m^2  S_TLU=HydFcnParams.liftValve.spoolPosVector mm  orifice_area_TLU=HydFcnParams.liftValve.PtoAOrificeAreaVector mm^2  area=inf m^2  Cd=0.64  Re_c=150  smoothing_factor=0.01  pressure_recovery=false  S_vol_flow_TLU=[0, .002, .004, .007, .017] m  p_diff_TLU=[.3, .5, .7] MPa  vol_flow_TLU=1e-3 * [1.7e-05, 2e-05, 2.6e-05; .0035, .0045, .0053; .7, .9, 1.06; 1.96, 2.5, 3; 6, 7.7, 9.13] m^3/s
      settings: InternalSimscapePortConfiguration="{\"Bottom\":[],\"Left\":[{\"id\":\"A\",\"label\":\"A\",\"type\":\"foundation.isothermal_liquid.isothermal_liquid\"}],\"Right\":[{\"id\":\"B\",\"label\":\"B\",\"type\":\"foundation.isothermal_liquid.isothermal_liquid\"}],\"Top\":[]}"
  Fixed Orifice Tilt : SimscapeFluids_lib/Isothermal Liquid/Valves & Orifices/Orifices/Orifice (IL)  orifice_type=foundation.enum.constant_variable.constant  constant_orifice_spec=fluids.isothermal_liquid.valves_orifices.orifices.enum.constant_orifice_spec.area  variable_orifice_spec=fluids.isothermal_liquid.valves_orifices.orifices.enum.orifice_spec.linear  orifice_area_constant=HydFcnParams.flowDivider.tiltFixedOrificeArea mm^2  p_diff_TLU_constant=[-4, -3, -2, -1, -.5, 0, .5, 1, 2, 3, 4] MPa  vol_flow_TLU_constant=[-2.44, -2.12, -1.68, -1.22, -.84, 0, .85, 1.21, 1.7, 2.09, 2.41] .* 1e-3 m^3/s  S_min=0 m  del_S=5e-3 m  open_orientation=fluids.isothermal_liquid.valves_orifices.orifices.enum.orifice_orientation.positive  area_max=HydFcnParams.flowDivider.tiltMaxOrificeArea mm^2  area_leak=1e-10 m^2  S_TLU=HydFcnParams.liftValve.spoolPosVector mm  orifice_area_TLU=HydFcnParams.liftValve.PtoAOrificeAreaVector mm^2  area=inf m^2  Cd=0.64  Re_c=150  smoothing_factor=0.01  pressure_recovery=false  S_vol_flow_TLU=[0, .002, .004, .007, .017] m  p_diff_TLU=[.3, .5, .7] MPa  vol_flow_TLU=1e-3 * [1.7e-05, 2e-05, 2.6e-05; .0035, .0045, .0053; .7, .9, 1.06; 1.96, 2.5, 3; 6, 7.7, 9.13] m^3/s
      settings: InternalSimscapePortConfiguration="{\"Bottom\":[],\"Left\":[{\"id\":\"A\",\"label\":\"A\",\"type\":\"foundation.isothermal_liquid.isothermal_liquid\"}],\"Right\":[{\"id\":\"B\",\"label\":\"B\",\"type\":\"foundation.isothermal_liquid.isothermal_liquid\"}],\"Top\":[]}"
  Variable Orifice Lift : SimscapeFluids_lib/Isothermal Liquid/Valves & Orifices/Orifices/Orifice (IL)  orifice_type=foundation.enum.constant_variable.variable  constant_orifice_spec=fluids.isothermal_liquid.valves_orifices.orifices.enum.constant_orifice_spec.area  variable_orifice_spec=fluids.isothermal_liquid.valves_orifices.orifices.enum.orifice_spec.table1D_area_opening  orifice_area_constant=1e-3 m^2  p_diff_TLU_constant=[-4, -3, -2, -1, -.5, 0, .5, 1, 2, 3, 4] MPa  vol_flow_TLU_constant=[-2.44, -2.12, -1.68, -1.22, -.84, 0, .85, 1.21, 1.7, 2.09, 2.41] .* 1e-3 m^3/s  S_min=0 m  del_S=5e-3 m  open_orientation=fluids.isothermal_liquid.valves_orifices.orifices.enum.orifice_orientation.positive  area_max=HydFcnParams.flowDivider.tiltMaxOrificeArea mm^2  area_leak=1e-10 m^2  S_TLU=HydFcnParams.flowDivider.liftSpoolVec mm  orifice_area_TLU=HydFcnParams.flowDivider.liftVarOrificeArea mm^2  area=inf m^2  Cd=0.64  Re_c=150  smoothing_factor=0.01  pressure_recovery=false  S_vol_flow_TLU=[0, .002, .004, .007, .017] m  p_diff_TLU=[.3, .5, .7] MPa  vol_flow_TLU=1e-3 * [1.7e-05, 2e-05, 2.6e-05; .0035, .0045, .0053; .7, .9, 1.06; 1.96, 2.5, 3; 6, 7.7, 9.13] m^3/s
      settings: InternalSimscapePortConfiguration="{\"Bottom\":[],\"Left\":[{\"id\":\"A\",\"label\":\"A\",\"type\":\"foundation.isothermal_liquid.isothermal_liquid\"},{\"id\":\"S\",\"label\":\"S\",\"type\":\"input\"}],\"Right\":[{\"id\":\"B\",\"label\":\"B\",\"type\":\"foundation.isothermal_liquid.isothermal_liquid\"}],\"Top\":[]}"
  Variable Orifice Tilt : SimscapeFluids_lib/Isothermal Liquid/Valves & Orifices/Orifices/Orifice (IL)  orifice_type=foundation.enum.constant_variable.variable  constant_orifice_spec=fluids.isothermal_liquid.valves_orifices.orifices.enum.constant_orifice_spec.area  variable_orifice_spec=fluids.isothermal_liquid.valves_orifices.orifices.enum.orifice_spec.table1D_area_opening  orifice_area_constant=1e-3 m^2  p_diff_TLU_constant=[-4, -3, -2, -1, -.5, 0, .5, 1, 2, 3, 4] MPa  vol_flow_TLU_constant=[-2.44, -2.12, -1.68, -1.22, -.84, 0, .85, 1.21, 1.7, 2.09, 2.41] .* 1e-3 m^3/s  S_min=0 m  del_S=5e-3 m  open_orientation=fluids.isothermal_liquid.valves_orifices.orifices.enum.orifice_orientation.positive  area_max=HydFcnParams.flowDivider.tiltMaxOrificeArea mm^2  area_leak=1e-10 m^2  S_TLU=HydFcnParams.flowDivider.tiltSpoolVec mm  orifice_area_TLU=HydFcnParams.flowDivider.tiltVarOrificeArea mm^2  area=inf m^2  Cd=0.64  Re_c=150  smoothing_factor=0.01  pressure_recovery=false  S_vol_flow_TLU=[0, .002, .004, .007, .017] m  p_diff_TLU=[.3, .5, .7] MPa  vol_flow_TLU=1e-3 * [1.7e-05, 2e-05, 2.6e-05; .0035, .0045, .0053; .7, .9, 1.06; 1.96, 2.5, 3; 6, 7.7, 9.13] m^3/s
      settings: InternalSimscapePortConfiguration="{\"Bottom\":[],\"Left\":[{\"id\":\"A\",\"label\":\"A\",\"type\":\"foundation.isothermal_liquid.isothermal_liquid\"},{\"id\":\"S\",\"label\":\"S\",\"type\":\"input\"}],\"Right\":[{\"id\":\"B\",\"label\":\"B\",\"type\":\"foundation.isothermal_liquid.isothermal_liquid\"}],\"Top\":[]}"
  P : PMIOPort  Side=Left
  Lift : PMIOPort  Port=2  Side=Right
  Tilt : PMIOPort  Port=3  Side=Right
  connections:
  Double-Acting Servo Valve Actuator (IL)/RConn1 -- Variable Orifice Tilt/LConn2 -- Variable Orifice Lift/LConn2
  Fixed Orifice Tilt/RConn1 -- Double-Acting Servo Valve Actuator (IL)/LConn1 -- Variable Orifice Tilt/LConn1
  Fixed Orifice Lift/RConn1 -- Double-Acting Servo Valve Actuator (IL)/LConn2 -- Variable Orifice Lift/LConn1
  Variable Orifice Lift/RConn1 -- Lift/RConn1
  Tilt/RConn1 -- Variable Orifice Tilt/RConn1
  P/RConn1 -- Fixed Orifice Tilt/LConn1 -- Fixed Orifice Lift/LConn1
